simulink model "r2_b8a4x128f_4gbe"  (R2012b)
settings: Solver=VariableStepDiscrete  SolverMode=SingleTasking  StartTime=0.0  StopTime=1  RelTol=1e-3
undefined symbols (not defined in the file): fft_stages, n_ants, n_bits_xengs
libraries: xbsIndex_r4 x21845, casper_library_misc x157, xbsReplacements_r4 x24, casper_library_communications x8, casper_library_delays x8, xps_library x5
(part 15 of 182)

== system r2_b8a4x128f_4gbe/latch0 ==
  reset : Inport
  gbe_down : Inport  Port=2
  rx_dest_err : Inport  Port=3
  feng_rx_err : Inport  Port=4
  fft_err : Inport  Port=5
  feng_qdr_err : Inport  Port=6
  feng_chk_err : Inport  Port=7
  adc_over : Inport  Port=8
  noise_diode_en : Inport  Port=9
  vacc_err : Inport  Port=10
  rx_bad_pkt : Inport  Port=11
  rx_bad_frame : Inport  Port=12
  tx_over : Inport  Port=13
  xeng_bad_dat : Inport  Port=14
  pack_err : Inport  Port=15
  rx : Inport  Port=16
  tx : Inport  Port=17
  flush : Inport  Port=18
  Delay{,1..16,33} (18 alike) : xbsIndex_r4/Delay  rst=off  infoeditControl=Selection of Reset will increase slice count due to use of real FFs and instead of SRLs  en=off  latency=1  dbl_ovrd=off  reg_retiming=off  block_type=delay
  Delay{17..32,34} (17 alike) : xbsIndex_r4/Delay  rst=on  infoeditControl=Selection of Reset will increase slice count due to use of real FFs and instead of SRLs  en=on  latency=1  dbl_ovrd=off  reg_retiming=on  block_type=delay
  Subsystem6 : Subsystem
  gbe_down_reg : Outport
  rx_dest_err_reg : Outport  Port=2
  feng_rx_err_reg : Outport  Port=3
  fft_err_reg : Outport  Port=4
  feng_qdr_err_reg : Outport  Port=5
  feng_chk_err_reg : Outport  Port=6
  adc_over_reg : Outport  Port=7
  noise_diode_en_reg : Outport  Port=8
  vacc_err_reg : Outport  Port=9
  rx_bad_pkt_reg : Outport  Port=10
  rx_bad_frame_reg : Outport  Port=11
  tx_over_reg : Outport  Port=12
  xeng_bad_dat_reg : Outport  Port=13
  pack_err_reg : Outport  Port=14
  rx_reg : Outport  Port=15
  tx_reg : Outport  Port=16
  data_bad : Outport  Port=17
  error : Outport  Port=18
  flush_reg : Outport  Port=19
  wires:
  rx_bad_pkt/1 -> Delay10/1
  pack_err/1 -> Delay14/1
  xeng_bad_dat/1 -> Delay13/1
  tx_over/1 -> Delay12/1
  rx_bad_frame/1 -> Delay11/1
  vacc_err/1 -> Delay9/1
  noise_diode_en/1 -> Delay8/1
  adc_over/1 -> Delay7/1
  feng_chk_err/1 -> Delay6/1
  feng_qdr_err/1 -> Delay5/1
  Subsystem6/2(err) -> error/1
  Subsystem6/1(data_in_bad) -> data_bad/1
  fft_err/1 -> Delay4/1
  feng_rx_err/1 -> Delay3/1
  rx_dest_err/1 -> Delay2/1
  gbe_down/1 -> Delay1/1
  reset/1 -> Delay/1
  Delay28/1 -> tx_over_reg/1
  Delay27/1 -> rx_bad_frame_reg/1
  Delay26/1 -> rx_bad_pkt_reg/1
  Delay25/1 -> vacc_err_reg/1
  Delay24/1 -> noise_diode_en_reg/1
  Delay23/1 -> adc_over_reg/1
  Delay22/1 -> feng_chk_err_reg/1
  Delay21/1 -> feng_qdr_err_reg/1
  Delay20/1 -> fft_err_reg/1
  Delay19/1 -> feng_rx_err_reg/1
  Delay17/1 -> gbe_down_reg/1
  Delay18/1 -> rx_dest_err_reg/1
  rx/1 -> Delay15/1
  Delay31/1 -> rx_reg/1
  tx/1 -> Delay16/1
  Delay32/1 -> tx_reg/1
  Delay/1 -> Delay17/2, Delay18/2, Delay19/2, Delay20/2, Delay21/2, Delay22/2, Delay23/2, Delay24/2, Delay25/2, Delay26/2, Delay27/2, Delay28/2, Delay29/2, Delay30/2, Delay34/2, Delay32/2, Delay31/2
  Delay1/1 -> Subsystem6/1(gbe_down), Delay17/3, Delay17/1
  Delay2/1 -> Delay18/3, Delay18/1, Subsystem6/2(rx_dest_err)
  Delay3/1 -> Delay19/3, Delay19/1, Subsystem6/3(feng_rx_err)
  Delay4/1 -> Delay20/1, Delay20/3, Subsystem6/4(fft_err)
  Delay7/1 -> Delay23/1, Delay23/3, Subsystem6/7(adc_over)
  Delay6/1 -> Delay22/1, Delay22/3, Subsystem6/6(feng_chk_err)
  Delay5/1 -> Delay21/3, Delay21/1, Subsystem6/5(feng_qdr_err)
  Delay11/1 -> Delay27/3, Delay27/1, Subsystem6/10(rx_bad_frame)
  Delay15/1 -> Delay31/1, Delay31/3
  Delay9/1 -> Delay25/3, Delay25/1, Subsystem6/8(vacc_err)
  Delay8/1 -> Delay24/1, Delay24/3
  Delay10/1 -> Delay26/1, Delay26/3, Subsystem6/9(rx_bad_pkt)
  Delay12/1 -> Delay28/1, Delay28/3, Subsystem6/11(tx_over)
  Delay13/1 -> Delay29/1, Delay29/3, Subsystem6/12(xeng_bad_dat)
  Delay14/1 -> Delay30/3, Delay30/1, Subsystem6/13(pack_err)
  Delay16/1 -> Delay32/3, Delay32/1
  Delay29/1 -> xeng_bad_dat_reg/1
  Delay30/1 -> pack_err_reg/1
  flush/1 -> Delay33/1
  Delay33/1 -> Delay34/3, Delay34/1
  Delay34/1 -> flush_reg/1

== system r2_b8a4x128f_4gbe/latch1 ==
  reset : Inport
  gbe_down : Inport  Port=2
  rx_dest_err : Inport  Port=3
  feng_rx_err : Inport  Port=4
  fft_err : Inport  Port=5
  feng_qdr_err : Inport  Port=6
  feng_chk_err : Inport  Port=7
  adc_over : Inport  Port=8
  noise_diode_en : Inport  Port=9
  vacc_err : Inport  Port=10
  rx_bad_pkt : Inport  Port=11
  rx_bad_frame : Inport  Port=12
  tx_over : Inport  Port=13
  xeng_bad_dat : Inport  Port=14
  pack_err : Inport  Port=15
  rx : Inport  Port=16
  tx : Inport  Port=17
  flush : Inport  Port=18
  Delay{,1..16,33} (18 alike) : xbsIndex_r4/Delay  rst=off  infoeditControl=Selection of Reset will increase slice count due to use of real FFs and instead of SRLs  en=off  latency=1  dbl_ovrd=off  reg_retiming=off  block_type=delay
  Delay{17..32,34} (17 alike) : xbsIndex_r4/Delay  rst=on  infoeditControl=Selection of Reset will increase slice count due to use of real FFs and instead of SRLs  en=on  latency=1  dbl_ovrd=off  reg_retiming=on  block_type=delay
  Subsystem6 : Subsystem
  gbe_down_reg : Outport
  rx_dest_err_reg : Outport  Port=2
  feng_rx_err_reg : Outport  Port=3
  fft_err_reg : Outport  Port=4
  feng_qdr_err_reg : Outport  Port=5
  feng_chk_err_reg : Outport  Port=6
  adc_over_reg : Outport  Port=7
  noise_diode_en_reg : Outport  Port=8
  vacc_err_reg : Outport  Port=9
  rx_bad_pkt_reg : Outport  Port=10
  rx_bad_frame_reg : Outport  Port=11
  tx_over_reg : Outport  Port=12
  xeng_bad_dat_reg : Outport  Port=13
  pack_err_reg : Outport  Port=14
  rx_reg : Outport  Port=15
  tx_reg : Outport  Port=16
  data_bad : Outport  Port=17
  error : Outport  Port=18
  flush_reg : Outport  Port=19
  wires:
  Delay34/1 -> flush_reg/1
  Delay33/1 -> Delay34/1, Delay34/3
  flush/1 -> Delay33/1
  Delay30/1 -> pack_err_reg/1
  Delay29/1 -> xeng_bad_dat_reg/1
  Delay16/1 -> Delay32/1, Delay32/3
  Delay14/1 -> Subsystem6/13(pack_err), Delay30/1, Delay30/3
  Delay13/1 -> Subsystem6/12(xeng_bad_dat), Delay29/3, Delay29/1
  Delay12/1 -> Subsystem6/11(tx_over), Delay28/3, Delay28/1
  Delay10/1 -> Subsystem6/9(rx_bad_pkt), Delay26/3, Delay26/1
  Delay8/1 -> Delay24/3, Delay24/1
  Delay9/1 -> Subsystem6/8(vacc_err), Delay25/1, Delay25/3
  Delay15/1 -> Delay31/3, Delay31/1
  Delay11/1 -> Subsystem6/10(rx_bad_frame), Delay27/1, Delay27/3
  Delay5/1 -> Subsystem6/5(feng_qdr_err), Delay21/1, Delay21/3
  Delay6/1 -> Subsystem6/6(feng_chk_err), Delay22/3, Delay22/1
  Delay7/1 -> Subsystem6/7(adc_over), Delay23/3, Delay23/1
  Delay4/1 -> Subsystem6/4(fft_err), Delay20/3, Delay20/1
  Delay3/1 -> Subsystem6/3(feng_rx_err), Delay19/1, Delay19/3
  Delay2/1 -> Subsystem6/2(rx_dest_err), Delay18/1, Delay18/3
  Delay1/1 -> Delay17/1, Delay17/3, Subsystem6/1(gbe_down)
  Delay/1 -> Delay31/2, Delay32/2, Delay34/2, Delay30/2, Delay29/2, Delay28/2, Delay27/2, Delay26/2, Delay25/2, Delay24/2, Delay23/2, Delay22/2, Delay21/2, Delay20/2, Delay19/2, Delay18/2, Delay17/2
  Delay32/1 -> tx_reg/1
  tx/1 -> Delay16/1
  Delay31/1 -> rx_reg/1
  rx/1 -> Delay15/1
  Delay18/1 -> rx_dest_err_reg/1
  Delay17/1 -> gbe_down_reg/1
  Delay19/1 -> feng_rx_err_reg/1
  Delay20/1 -> fft_err_reg/1
  Delay21/1 -> feng_qdr_err_reg/1
  Delay22/1 -> feng_chk_err_reg/1
  Delay23/1 -> adc_over_reg/1
  Delay24/1 -> noise_diode_en_reg/1
  Delay25/1 -> vacc_err_reg/1
  Delay26/1 -> rx_bad_pkt_reg/1
  Delay27/1 -> rx_bad_frame_reg/1
  Delay28/1 -> tx_over_reg/1
  reset/1 -> Delay/1
  gbe_down/1 -> Delay1/1
  rx_dest_err/1 -> Delay2/1
  feng_rx_err/1 -> Delay3/1
  fft_err/1 -> Delay4/1
  Subsystem6/1(data_in_bad) -> data_bad/1
  Subsystem6/2(err) -> error/1
  feng_qdr_err/1 -> Delay5/1
  feng_chk_err/1 -> Delay6/1
  adc_over/1 -> Delay7/1
  noise_diode_en/1 -> Delay8/1
  vacc_err/1 -> Delay9/1
  rx_bad_frame/1 -> Delay11/1
  tx_over/1 -> Delay12/1
  xeng_bad_dat/1 -> Delay13/1
  pack_err/1 -> Delay14/1
  rx_bad_pkt/1 -> Delay10/1

== system r2_b8a4x128f_4gbe/latch2 ==
  reset : Inport
  gbe_down : Inport  Port=2
  rx_dest_err : Inport  Port=3
  feng_rx_err : Inport  Port=4
  fft_err : Inport  Port=5
  feng_qdr_err : Inport  Port=6
  feng_chk_err : Inport  Port=7
  adc_over : Inport  Port=8
  noise_diode_en : Inport  Port=9
  vacc_err : Inport  Port=10
  rx_bad_pkt : Inport  Port=11
  rx_bad_frame : Inport  Port=12
  tx_over : Inport  Port=13
  xeng_bad_dat : Inport  Port=14
  pack_err : Inport  Port=15
  rx : Inport  Port=16
  tx : Inport  Port=17
  flush : Inport  Port=18
  Delay{,1..16,33} (18 alike) : xbsIndex_r4/Delay  rst=off  infoeditControl=Selection of Reset will increase slice count due to use of real FFs and instead of SRLs  en=off  latency=1  dbl_ovrd=off  reg_retiming=off  block_type=delay
  Delay{17..32,34} (17 alike) : xbsIndex_r4/Delay  rst=on  infoeditControl=Selection of Reset will increase slice count due to use of real FFs and instead of SRLs  en=on  latency=1  dbl_ovrd=off  reg_retiming=on  block_type=delay
  Subsystem6 : Subsystem
  gbe_down_reg : Outport
  rx_dest_err_reg : Outport  Port=2
  feng_rx_err_reg : Outport  Port=3
  fft_err_reg : Outport  Port=4
  feng_qdr_err_reg : Outport  Port=5
  feng_chk_err_reg : Outport  Port=6
  adc_over_reg : Outport  Port=7
  noise_diode_en_reg : Outport  Port=8
  vacc_err_reg : Outport  Port=9
  rx_bad_pkt_reg : Outport  Port=10
  rx_bad_frame_reg : Outport  Port=11
  tx_over_reg : Outport  Port=12
  xeng_bad_dat_reg : Outport  Port=13
  pack_err_reg : Outport  Port=14
  rx_reg : Outport  Port=15
  tx_reg : Outport  Port=16
  data_bad : Outport  Port=17
  error : Outport  Port=18
  flush_reg : Outport  Port=19
  wires:
  rx_bad_pkt/1 -> Delay10/1
  pack_err/1 -> Delay14/1
  xeng_bad_dat/1 -> Delay13/1
  tx_over/1 -> Delay12/1
  rx_bad_frame/1 -> Delay11/1
  vacc_err/1 -> Delay9/1
  noise_diode_en/1 -> Delay8/1
  adc_over/1 -> Delay7/1
  feng_chk_err/1 -> Delay6/1
  feng_qdr_err/1 -> Delay5/1
  Subsystem6/2(err) -> error/1
  Subsystem6/1(data_in_bad) -> data_bad/1
  fft_err/1 -> Delay4/1
  feng_rx_err/1 -> Delay3/1
  rx_dest_err/1 -> Delay2/1
  gbe_down/1 -> Delay1/1
  reset/1 -> Delay/1
  Delay28/1 -> tx_over_reg/1
  Delay27/1 -> rx_bad_frame_reg/1
  Delay26/1 -> rx_bad_pkt_reg/1
  Delay25/1 -> vacc_err_reg/1
  Delay24/1 -> noise_diode_en_reg/1
  Delay23/1 -> adc_over_reg/1
  Delay22/1 -> feng_chk_err_reg/1
  Delay21/1 -> feng_qdr_err_reg/1
  Delay20/1 -> fft_err_reg/1
  Delay19/1 -> feng_rx_err_reg/1
  Delay17/1 -> gbe_down_reg/1
  Delay18/1 -> rx_dest_err_reg/1
  rx/1 -> Delay15/1
  Delay31/1 -> rx_reg/1
  tx/1 -> Delay16/1
  Delay32/1 -> tx_reg/1
  Delay/1 -> Delay17/2, Delay18/2, Delay19/2, Delay20/2, Delay21/2, Delay22/2, Delay23/2, Delay24/2, Delay25/2, Delay26/2, Delay27/2, Delay28/2, Delay29/2, Delay30/2, Delay34/2, Delay32/2, Delay31/2
  Delay1/1 -> Subsystem6/1(gbe_down), Delay17/3, Delay17/1
  Delay2/1 -> Delay18/3, Delay18/1, Subsystem6/2(rx_dest_err)
  Delay3/1 -> Delay19/3, Delay19/1, Subsystem6/3(feng_rx_err)
  Delay4/1 -> Delay20/1, Delay20/3, Subsystem6/4(fft_err)
  Delay7/1 -> Delay23/1, Delay23/3, Subsystem6/7(adc_over)
  Delay6/1 -> Delay22/1, Delay22/3, Subsystem6/6(feng_chk_err)
  Delay5/1 -> Delay21/3, Delay21/1, Subsystem6/5(feng_qdr_err)
  Delay11/1 -> Delay27/3, Delay27/1, Subsystem6/10(rx_bad_frame)
  Delay15/1 -> Delay31/1, Delay31/3
  Delay9/1 -> Delay25/3, Delay25/1, Subsystem6/8(vacc_err)
  Delay8/1 -> Delay24/1, Delay24/3
  Delay10/1 -> Delay26/1, Delay26/3, Subsystem6/9(rx_bad_pkt)
  Delay12/1 -> Delay28/1, Delay28/3, Subsystem6/11(tx_over)
  Delay13/1 -> Delay29/1, Delay29/3, Subsystem6/12(xeng_bad_dat)
  Delay14/1 -> Delay30/3, Delay30/1, Subsystem6/13(pack_err)
  Delay16/1 -> Delay32/3, Delay32/1
  Delay29/1 -> xeng_bad_dat_reg/1
  Delay30/1 -> pack_err_reg/1
  flush/1 -> Delay33/1
  Delay33/1 -> Delay34/3, Delay34/1
  Delay34/1 -> flush_reg/1

== system r2_b8a4x128f_4gbe/latch3 ==
  reset : Inport
  gbe_down : Inport  Port=2
  rx_dest_err : Inport  Port=3
  feng_rx_err : Inport  Port=4
  fft_err : Inport  Port=5
  feng_qdr_err : Inport  Port=6
  feng_chk_err : Inport  Port=7
  adc_over : Inport  Port=8
  noise_diode_en : Inport  Port=9
  vacc_err : Inport  Port=10
  rx_bad_pkt : Inport  Port=11
  rx_bad_frame : Inport  Port=12
  tx_over : Inport  Port=13
  xeng_bad_dat : Inport  Port=14
  pack_err : Inport  Port=15
  rx : Inport  Port=16
  tx : Inport  Port=17
  flush : Inport  Port=18
  Delay{,1..16,33} (18 alike) : xbsIndex_r4/Delay  rst=off  infoeditControl=Selection of Reset will increase slice count due to use of real FFs and instead of SRLs  en=off  latency=1  dbl_ovrd=off  reg_retiming=off  block_type=delay
  Delay{17..32,34} (17 alike) : xbsIndex_r4/Delay  rst=on  infoeditControl=Selection of Reset will increase slice count due to use of real FFs and instead of SRLs  en=on  latency=1  dbl_ovrd=off  reg_retiming=on  block_type=delay
  Subsystem6 : Subsystem
  gbe_down_reg : Outport
  rx_dest_err_reg : Outport  Port=2
  feng_rx_err_reg : Outport  Port=3
  fft_err_reg : Outport  Port=4
  feng_qdr_err_reg : Outport  Port=5
  feng_chk_err_reg : Outport  Port=6
  adc_over_reg : Outport  Port=7
  noise_diode_en_reg : Outport  Port=8
  vacc_err_reg : Outport  Port=9
  rx_bad_pkt_reg : Outport  Port=10
  rx_bad_frame_reg : Outport  Port=11
  tx_over_reg : Outport  Port=12
  xeng_bad_dat_reg : Outport  Port=13
  pack_err_reg : Outport  Port=14
  rx_reg : Outport  Port=15
  tx_reg : Outport  Port=16
  data_bad : Outport  Port=17
  error : Outport  Port=18
  flush_reg : Outport  Port=19
  wires:
  Delay34/1 -> flush_reg/1
  Delay33/1 -> Delay34/1, Delay34/3
  flush/1 -> Delay33/1
  Delay30/1 -> pack_err_reg/1
  Delay29/1 -> xeng_bad_dat_reg/1
  Delay16/1 -> Delay32/1, Delay32/3
  Delay14/1 -> Subsystem6/13(pack_err), Delay30/1, Delay30/3
  Delay13/1 -> Subsystem6/12(xeng_bad_dat), Delay29/3, Delay29/1
  Delay12/1 -> Subsystem6/11(tx_over), Delay28/3, Delay28/1
  Delay10/1 -> Subsystem6/9(rx_bad_pkt), Delay26/3, Delay26/1
  Delay8/1 -> Delay24/3, Delay24/1
  Delay9/1 -> Subsystem6/8(vacc_err), Delay25/1, Delay25/3
  Delay15/1 -> Delay31/3, Delay31/1
  Delay11/1 -> Subsystem6/10(rx_bad_frame), Delay27/1, Delay27/3
  Delay5/1 -> Subsystem6/5(feng_qdr_err), Delay21/1, Delay21/3
  Delay6/1 -> Subsystem6/6(feng_chk_err), Delay22/3, Delay22/1
  Delay7/1 -> Subsystem6/7(adc_over), Delay23/3, Delay23/1
  Delay4/1 -> Subsystem6/4(fft_err), Delay20/3, Delay20/1
  Delay3/1 -> Subsystem6/3(feng_rx_err), Delay19/1, Delay19/3
  Delay2/1 -> Subsystem6/2(rx_dest_err), Delay18/1, Delay18/3
  Delay1/1 -> Delay17/1, Delay17/3, Subsystem6/1(gbe_down)
  Delay/1 -> Delay31/2, Delay32/2, Delay34/2, Delay30/2, Delay29/2, Delay28/2, Delay27/2, Delay26/2, Delay25/2, Delay24/2, Delay23/2, Delay22/2, Delay21/2, Delay20/2, Delay19/2, Delay18/2, Delay17/2
  Delay32/1 -> tx_reg/1
  tx/1 -> Delay16/1
  Delay31/1 -> rx_reg/1
  rx/1 -> Delay15/1
  Delay18/1 -> rx_dest_err_reg/1
  Delay17/1 -> gbe_down_reg/1
  Delay19/1 -> feng_rx_err_reg/1
  Delay20/1 -> fft_err_reg/1
  Delay21/1 -> feng_qdr_err_reg/1
  Delay22/1 -> feng_chk_err_reg/1
  Delay23/1 -> adc_over_reg/1
  Delay24/1 -> noise_diode_en_reg/1
  Delay25/1 -> vacc_err_reg/1
  Delay26/1 -> rx_bad_pkt_reg/1
  Delay27/1 -> rx_bad_frame_reg/1
  Delay28/1 -> tx_over_reg/1
  reset/1 -> Delay/1
  gbe_down/1 -> Delay1/1
  rx_dest_err/1 -> Delay2/1
  feng_rx_err/1 -> Delay3/1
  fft_err/1 -> Delay4/1
  Subsystem6/1(data_in_bad) -> data_bad/1
  Subsystem6/2(err) -> error/1
  feng_qdr_err/1 -> Delay5/1
  feng_chk_err/1 -> Delay6/1
  adc_over/1 -> Delay7/1
  noise_diode_en/1 -> Delay8/1
  vacc_err/1 -> Delay9/1
  rx_bad_frame/1 -> Delay11/1
  tx_over/1 -> Delay12/1
  xeng_bad_dat/1 -> Delay13/1
  pack_err/1 -> Delay14/1
  rx_bad_pkt/1 -> Delay10/1

== system r2_b8a4x128f_4gbe/miss_cnt0 ==
  Convert : xbsIndex_r4/Convert  gui_display_data_type=Fixed-point  arith_type=Unsigned  n_bits=32  bin_pt=0  float_type=Single  exp_bits=8  fraction_bits=24  quantization=Truncate  overflow=Wrap  en=off  latency=0  dbl_ovrd=off  pipeline=off  block_type=convert
  Counter1 : xbsIndex_r4/Counter  cnt_type=Free Running  cnt_to=1023  operation=Up  start_count=0  cnt_by_val=1  arith_type=Unsigned  n_bits=16  bin_pt=0  load_pin=off  rst=on  en=on  explicit_period=on  period=1  dbl_ovrd=off  use_behavioral_HDL=on  implementation=Fabric  use_rpm=on  block_type=counter
      settings: xl_area=[0, 0, 0, 0, 0, 0, 0]
  Delay1 : Subsystem  AncestorBlock=casper_library_delays/pipeline  mask(pipeline){latency=2}
      mask help:
      | An explicitly laid-out delay line to avoid mapping to SRL16s
      | for use in pipelining to help achieve timing closure.
      mask init:
      | pipeline_init(gcb,'latency',latency);
      settings: AttributesFormatString=Latency = %<latency>
      mask Display:
      | port_label('input', 1, 'd');
      | port_label('output', 1, 'q');
      | disp(['Z^-', num2str(latency)]);
  Delay10 : Subsystem  AncestorBlock=casper_library_delays/pipeline  mask(pipeline){latency=2}
      mask help:
      | An explicitly laid-out delay line to avoid mapping to SRL16s
      | for use in pipelining to help achieve timing closure.
      mask init:
      | pipeline_init(gcb,'latency',latency);
      settings: AttributesFormatString=Latency = %<latency>
      mask Display:
      | port_label('input', 1, 'd');
      | port_label('output', 1, 'q');
      | disp(['Z^-', num2str(latency)]);
  Delay11 : Subsystem  AncestorBlock=casper_library_delays/pipeline  mask(pipeline){latency=2}
      mask help:
      | An explicitly laid-out delay line to avoid mapping to SRL16s
      | for use in pipelining to help achieve timing closure.
      mask init:
      | pipeline_init(gcb,'latency',latency);
      settings: AttributesFormatString=Latency = %<latency>
      mask Display:
      | port_label('input', 1, 'd');
      | port_label('output', 1, 'q');
      | disp(['Z^-', num2str(latency)]);
  Delay12 : Subsystem  AncestorBlock=casper_library_delays/pipeline  mask(pipeline){latency=2}
      mask help:
      | An explicitly laid-out delay line to avoid mapping to SRL16s
      | for use in pipelining to help achieve timing closure.
      mask init:
      | pipeline_init(gcb,'latency',latency);
      settings: AttributesFormatString=Latency = %<latency>
      mask Display:
      | port_label('input', 1, 'd');
      | port_label('output', 1, 'q');
      | disp(['Z^-', num2str(latency)]);
  Delay13 : Subsystem  AncestorBlock=casper_library_delays/pipeline  mask(pipeline){latency=2}
      mask help:
      | An explicitly laid-out delay line to avoid mapping to SRL16s
      | for use in pipelining to help achieve timing closure.
      mask init:
      | pipeline_init(gcb,'latency',latency);
      settings: AttributesFormatString=Latency = %<latency>
      mask Display:
      | port_label('input', 1, 'd');
      | port_label('output', 1, 'q');
      | disp(['Z^-', num2str(latency)]);
  Delay14 : Subsystem  AncestorBlock=casper_library_delays/pipeline  mask(pipeline){latency=2}
      mask help:
      | An explicitly laid-out delay line to avoid mapping to SRL16s
      | for use in pipelining to help achieve timing closure.
      mask init:
      | pipeline_init(gcb,'latency',latency);
      settings: AttributesFormatString=Latency = %<latency>
      mask Display:
      | port_label('input', 1, 'd');
      | port_label('output', 1, 'q');
      | disp(['Z^-', num2str(latency)]);
  Delay15 : Subsystem  AncestorBlock=casper_library_delays/pipeline  mask(pipeline){latency=2}
      mask help:
      | An explicitly laid-out delay line to avoid mapping to SRL16s
      | for use in pipelining to help achieve timing closure.
      mask init:
      | pipeline_init(gcb,'latency',latency);
      settings: AttributesFormatString=Latency = %<latency>
      mask Display:
      | port_label('input', 1, 'd');
      | port_label('output', 1, 'q');
      | disp(['Z^-', num2str(latency)]);
  Delay2 : Subsystem  AncestorBlock=casper_library_delays/pipeline  mask(pipeline){latency=2}
      mask help:
      | An explicitly laid-out delay line to avoid mapping to SRL16s
      | for use in pipelining to help achieve timing closure.
      mask init:
      | pipeline_init(gcb,'latency',latency);
      settings: AttributesFormatString=Latency = %<latency>
      mask Display:
      | port_label('input', 1, 'd');
      | port_label('output', 1, 'q');
      | disp(['Z^-', num2str(latency)]);
  Delay3 : Subsystem  AncestorBlock=casper_library_delays/pipeline  mask(pipeline){latency=2}
      mask help:
      | An explicitly laid-out delay line to avoid mapping to SRL16s
      | for use in pipelining to help achieve timing closure.
      mask init:
      | pipeline_init(gcb,'latency',latency);
      settings: AttributesFormatString=Latency = %<latency>
      mask Display:
      | port_label('input', 1, 'd');
      | port_label('output', 1, 'q');
      | disp(['Z^-', num2str(latency)]);
  Delay4 : Subsystem  AncestorBlock=casper_library_delays/pipeline  mask(pipeline){latency=1}
      mask help:
      | An explicitly laid-out delay line to avoid mapping to SRL16s
      | for use in pipelining to help achieve timing closure.
      mask init:
      | pipeline_init(gcb,'latency',latency);
      settings: AttributesFormatString=Latency = %<latency>
      mask Display:
      | port_label('input', 1, 'd');
      | port_label('output', 1, 'q');
      | disp(['Z^-', num2str(latency)]);
  Delay5 : Subsystem  AncestorBlock=casper_library_delays/pipeline  mask(pipeline){latency=2}
      mask help:
      | An explicitly laid-out delay line to avoid mapping to SRL16s
      | for use in pipelining to help achieve timing closure.
      mask init:
      | pipeline_init(gcb,'latency',latency);
      settings: AttributesFormatString=Latency = %<latency>
      mask Display:
      | port_label('input', 1, 'd');
      | port_label('output', 1, 'q');
      | disp(['Z^-', num2str(latency)]);
  Delay6 : Subsystem  AncestorBlock=casper_library_delays/pipeline  mask(pipeline){latency=3}
      mask help:
      | An explicitly laid-out delay line to avoid mapping to SRL16s
      | for use in pipelining to help achieve timing closure.
      mask init:
      | pipeline_init(gcb,'latency',latency);
      settings: AttributesFormatString=Latency = %<latency>
      mask Display:
      | port_label('input', 1, 'd');
      | port_label('output', 1, 'q');
      | disp(['Z^-', num2str(latency)]);
  Delay7 : Subsystem  AncestorBlock=casper_library_delays/pipeline  mask(pipeline){latency=2}
      mask help:
      | An explicitly laid-out delay line to avoid mapping to SRL16s
      | for use in pipelining to help achieve timing closure.
      mask init:
      | pipeline_init(gcb,'latency',latency);
      settings: AttributesFormatString=Latency = %<latency>
      mask Display:
      | port_label('input', 1, 'd');
      | port_label('output', 1, 'q');
      | disp(['Z^-', num2str(latency)]);
  Delay8 : Subsystem  AncestorBlock=casper_library_delays/pipeline  mask(pipeline){latency=2}
      mask help:
      | An explicitly laid-out delay line to avoid mapping to SRL16s
      | for use in pipelining to help achieve timing closure.
      mask init:
      | pipeline_init(gcb,'latency',latency);
      settings: AttributesFormatString=Latency = %<latency>
      mask Display:
      | port_label('input', 1, 'd');
      | port_label('output', 1, 'q');
      | disp(['Z^-', num2str(latency)]);
  Delay9 : Subsystem  AncestorBlock=casper_library_delays/pipeline  mask(pipeline){latency=2}
      mask help:
      | An explicitly laid-out delay line to avoid mapping to SRL16s
      | for use in pipelining to help achieve timing closure.
      mask init:
      | pipeline_init(gcb,'latency',latency);
      settings: AttributesFormatString=Latency = %<latency>
      mask Display:
      | port_label('input', 1, 'd');
      | port_label('output', 1, 'q');
      | disp(['Z^-', num2str(latency)]);
  Delay96 : Subsystem  AncestorBlock=casper_library_delays/pipeline  mask(pipeline){latency=2}
      mask help:
      | An explicitly laid-out delay line to avoid mapping to SRL16s
      | for use in pipelining to help achieve timing closure.
      mask init:
      | pipeline_init(gcb,'latency',latency);
      settings: AttributesFormatString=Latency = %<latency>
      mask Display:
      | port_label('input', 1, 'd');
      | port_label('output', 1, 'q');
      | disp(['Z^-', num2str(latency)]);
  Delay97 : Subsystem  AncestorBlock=casper_library_delays/pipeline  mask(pipeline){latency=2}
      mask help:
      | An explicitly laid-out delay line to avoid mapping to SRL16s
      | for use in pipelining to help achieve timing closure.
      mask init:
      | pipeline_init(gcb,'latency',latency);
      settings: AttributesFormatString=Latency = %<latency>
      mask Display:
      | port_label('input', 1, 'd');
      | port_label('output', 1, 'q');
      | disp(['Z^-', num2str(latency)]);
  Delay98 : Subsystem  AncestorBlock=casper_library_delays/pipeline  mask(pipeline){latency=2}
      mask help:
      | An explicitly laid-out delay line to avoid mapping to SRL16s
      | for use in pipelining to help achieve timing closure.
      mask init:
      | pipeline_init(gcb,'latency',latency);
      settings: AttributesFormatString=Latency = %<latency>
      mask Display:
      | port_label('input', 1, 'd');
      | port_label('output', 1, 'q');
      | disp(['Z^-', num2str(latency)]);
  Logical{1..4} (4 alike) : xbsIndex_r4/Logical  logical_function=AND  inputs=2  en=off  latency=1  precision=Full  arith_type=Unsigned  n_bits=8  bin_pt=2  align_bp=on  dbl_ovrd=off  block_type=logical
      settings: xl_area=[0, 0, 0, 0, 0, 0, 0]
  Register : xbsIndex_r4/Register  init=0  rst=on  en=on  dbl_ovrd=off  block_type=register
  Slice : xbsIndex_r4/Slice  nbits=16  boolean_output=off  mode=Two Bit Locations  bit1=0  base1=MSB of Input  bit0=xeng_int_bits  base0=LSB of Input  dbl_ovrd=off  block_type=slice
      settings: infoedit="Extracts a given range of bits from each input sample and presents it at the output.  The output type is ordinarily unsigned with binary point at zero, but can be Boolean when the slice is one bit wide.<P><P>Hardware notes: In hardware this block costs nothing."  block_version=10.1.3
  ant_cnt : xbsIndex_r4/Counter  cnt_type=Free Running  cnt_to=1023  operation=Up  start_count=0  cnt_by_val=1  arith_type=Unsigned  n_bits=xeng_int_bits + n_ants_bits  bin_pt=0  load_pin=off  rst=on  en=on  explicit_period=on  period=1  dbl_ovrd=off  use_behavioral_HDL=on  implementation=Fabric  use_rpm=on  block_type=counter
      settings: xl_area=[0, 0, 0, 0, 0, 0, 0]
  sync_ctr1 : xbsIndex_r4/Counter  cnt_type=Free Running  cnt_to=1023  operation=Up  start_count=0  cnt_by_val=1  arith_type=Unsigned  n_bits=32  bin_pt=0  load_pin=off  rst=on  en=on  explicit_period=on  period=1  dbl_ovrd=off  use_behavioral_HDL=off  implementation=Fabric  use_rpm=on  block_type=counter
      settings: xl_area=[0, 0, 0, 0, 0, 0, 0]
  sync_ctr5 : xbsIndex_r4/Counter  cnt_type=Free Running  cnt_to=1023  operation=Up  start_count=0  cnt_by_val=1  arith_type=Unsigned  n_bits=16  bin_pt=0  load_pin=off  rst=on  en=on  explicit_period=on  period=1  dbl_ovrd=off  use_behavioral_HDL=on  implementation=Fabric  use_rpm=on  block_type=counter
      settings: xl_area=[0, 0, 0, 0, 0, 0, 0]
  sync_ctr6 : xbsIndex_r4/Counter  cnt_type=Free Running  cnt_to=1023  operation=Up  start_count=0  cnt_by_val=1  arith_type=Unsigned  n_bits=16  bin_pt=0  load_pin=off  rst=on  en=on  explicit_period=on  period=1  dbl_ovrd=off  use_behavioral_HDL=on  implementation=Fabric  use_rpm=on  block_type=counter
      settings: xl_area=[0, 0, 0, 0, 0, 0, 0]
  sync_ctr8 : xbsIndex_r4/Counter  cnt_type=Free Running  cnt_to=1023  operation=Up  start_count=0  cnt_by_val=1  arith_type=Unsigned  n_bits=32  bin_pt=0  load_pin=off  rst=on  en=on  explicit_period=on  period=1  dbl_ovrd=off  use_behavioral_HDL=off  implementation=Fabric  use_rpm=on  block_type=counter
      settings: xl_area=[0, 0, 0, 0, 0, 0, 0]
  spectr_cnt : Outport
  last_missed_ant : Outport  Port=2
  recv_ctr : Outport  Port=3
  recv_errctr : Outport  Port=4
  timeout_errctr : Outport  Port=5
  pktdisc_errctr : Outport  Port=6
  wires:
  Delay1/1(q) -> Register/2, Counter1/1
  Delay3/1(q) -> ant_cnt/2
  Delay2/1(q) -> Counter1/2, ant_cnt/1
  Counter1/1 -> Delay11/1(d)
  Register/1 -> Delay15/1(d)
  ant_cnt/1 -> Slice/1
  Slice/1 -> Register/1
  [reord_timeouterr0] -> Delay97/1(d)
  Logical3/1 -> sync_ctr6/2
  Delay96/1(q) -> sync_ctr1/1, sync_ctr5/1, sync_ctr6/1
  Delay97/1(q) -> Logical3/2
  [cnt_rst] -> Delay96/1(d)
  [reord_valid0] -> Delay98/1(d)
  Delay98/1(q) -> Logical2/1, Logical1/1, Logical3/1
  Logical1/1 -> sync_ctr5/2
  Delay8/1(q) -> Logical1/2
  [reord_pktdisc0] -> Delay8/1(d)
  sync_ctr8/1 -> Delay10/1(d)
  Logical4/1 -> sync_ctr8/2
  Delay12/1(q) -> sync_ctr8/1
  Delay13/1(q) -> Logical4/2
  [cnt_rst] -> Delay12/1(d)
  [reord_valid0] -> Delay14/1(d)
  Delay14/1(q) -> Logical4/1
  [reord_recv0] -> Delay13/1(d)
  sync_ctr6/1 -> Delay5/1(d)
  sync_ctr5/1 -> Delay6/1(d)
  sync_ctr1/1 -> Delay4/1(d)
  Delay4/1(q) -> recv_errctr/1
  Delay5/1(q) -> timeout_errctr/1
  Delay6/1(q) -> pktdisc_errctr/1
  Logical2/1 -> sync_ctr1/2
  Delay7/1(q) -> Logical2/2
  [reord_recverr0] -> Delay7/1(d)
  [cnt_rst] -> Delay1/1(d)
  [reord_sync0] -> Delay2/1(d)
  [reord_valid0] -> Delay3/1(d)
  [reord_recverr0] -> Delay9/1(d)
  Delay10/1(q) -> recv_ctr/1
  Delay11/1(q) -> spectr_cnt/1
  Delay15/1(q) -> Convert/1
  Convert/1 -> last_missed_ant/1
  Delay9/1(q) -> Register/3

== system r2_b8a4x128f_4gbe/miss_cnt1 ==
  Convert : xbsIndex_r4/Convert  gui_display_data_type=Fixed-point  arith_type=Unsigned  n_bits=32  bin_pt=0  float_type=Single  exp_bits=8  fraction_bits=24  quantization=Truncate  overflow=Wrap  en=off  latency=0  dbl_ovrd=off  pipeline=off  block_type=convert
  Counter1 : xbsIndex_r4/Counter  cnt_type=Free Running  cnt_to=1023  operation=Up  start_count=0  cnt_by_val=1  arith_type=Unsigned  n_bits=16  bin_pt=0  load_pin=off  rst=on  en=on  explicit_period=on  period=1  dbl_ovrd=off  use_behavioral_HDL=on  implementation=Fabric  use_rpm=on  block_type=counter
      settings: xl_area=[0, 0, 0, 0, 0, 0, 0]
  Delay1 : Subsystem  AncestorBlock=casper_library_delays/pipeline  mask(pipeline){latency=2}
      mask help:
      | An explicitly laid-out delay line to avoid mapping to SRL16s
      | for use in pipelining to help achieve timing closure.
      mask init:
      | pipeline_init(gcb,'latency',latency);
      settings: AttributesFormatString=Latency = %<latency>
      mask Display:
      | port_label('input', 1, 'd');
      | port_label('output', 1, 'q');
      | disp(['Z^-', num2str(latency)]);
  Delay10 : Subsystem  AncestorBlock=casper_library_delays/pipeline  mask(pipeline){latency=2}
      mask help:
      | An explicitly laid-out delay line to avoid mapping to SRL16s
      | for use in pipelining to help achieve timing closure.
      mask init:
      | pipeline_init(gcb,'latency',latency);
      settings: AttributesFormatString=Latency = %<latency>
      mask Display:
      | port_label('input', 1, 'd');
      | port_label('output', 1, 'q');
      | disp(['Z^-', num2str(latency)]);
  Delay11 : Subsystem  AncestorBlock=casper_library_delays/pipeline  mask(pipeline){latency=2}
      mask help:
      | An explicitly laid-out delay line to avoid mapping to SRL16s
      | for use in pipelining to help achieve timing closure.
      mask init:
      | pipeline_init(gcb,'latency',latency);
      settings: AttributesFormatString=Latency = %<latency>
      mask Display:
      | port_label('input', 1, 'd');
      | port_label('output', 1, 'q');
      | disp(['Z^-', num2str(latency)]);
  Delay12 : Subsystem  AncestorBlock=casper_library_delays/pipeline  mask(pipeline){latency=2}
      mask help:
      | An explicitly laid-out delay line to avoid mapping to SRL16s
      | for use in pipelining to help achieve timing closure.
      mask init:
      | pipeline_init(gcb,'latency',latency);
      settings: AttributesFormatString=Latency = %<latency>
      mask Display:
      | port_label('input', 1, 'd');
      | port_label('output', 1, 'q');
      | disp(['Z^-', num2str(latency)]);
  Delay13 : Subsystem  AncestorBlock=casper_library_delays/pipeline  mask(pipeline){latency=2}
      mask help:
      | An explicitly laid-out delay line to avoid mapping to SRL16s
      | for use in pipelining to help achieve timing closure.
      mask init:
      | pipeline_init(gcb,'latency',latency);
      settings: AttributesFormatString=Latency = %<latency>
      mask Display:
      | port_label('input', 1, 'd');
      | port_label('output', 1, 'q');
      | disp(['Z^-', num2str(latency)]);
  Delay14 : Subsystem  AncestorBlock=casper_library_delays/pipeline  mask(pipeline){latency=2}
      mask help:
      | An explicitly laid-out delay line to avoid mapping to SRL16s
      | for use in pipelining to help achieve timing closure.
      mask init:
      | pipeline_init(gcb,'latency',latency);
      settings: AttributesFormatString=Latency = %<latency>
      mask Display:
      | port_label('input', 1, 'd');
      | port_label('output', 1, 'q');
      | disp(['Z^-', num2str(latency)]);
  Delay15 : Subsystem  AncestorBlock=casper_library_delays/pipeline  mask(pipeline){latency=2}
      mask help:
      | An explicitly laid-out delay line to avoid mapping to SRL16s
      | for use in pipelining to help achieve timing closure.
      mask init:
      | pipeline_init(gcb,'latency',latency);
      settings: AttributesFormatString=Latency = %<latency>
      mask Display:
      | port_label('input', 1, 'd');
      | port_label('output', 1, 'q');
      | disp(['Z^-', num2str(latency)]);
  Delay2 : Subsystem  AncestorBlock=casper_library_delays/pipeline  mask(pipeline){latency=2}
      mask help:
      | An explicitly laid-out delay line to avoid mapping to SRL16s
      | for use in pipelining to help achieve timing closure.
      mask init:
      | pipeline_init(gcb,'latency',latency);
      settings: AttributesFormatString=Latency = %<latency>
      mask Display:
      | port_label('input', 1, 'd');
      | port_label('output', 1, 'q');
      | disp(['Z^-', num2str(latency)]);
  Delay3 : Subsystem  AncestorBlock=casper_library_delays/pipeline  mask(pipeline){latency=2}
      mask help:
      | An explicitly laid-out delay line to avoid mapping to SRL16s
      | for use in pipelining to help achieve timing closure.
      mask init:
      | pipeline_init(gcb,'latency',latency);
      settings: AttributesFormatString=Latency = %<latency>
      mask Display:
      | port_label('input', 1, 'd');
      | port_label('output', 1, 'q');
      | disp(['Z^-', num2str(latency)]);
  Delay4 : Subsystem  AncestorBlock=casper_library_delays/pipeline  mask(pipeline){latency=1}
      mask help:
      | An explicitly laid-out delay line to avoid mapping to SRL16s
      | for use in pipelining to help achieve timing closure.
      mask init:
      | pipeline_init(gcb,'latency',latency);
      settings: AttributesFormatString=Latency = %<latency>
      mask Display:
      | port_label('input', 1, 'd');
      | port_label('output', 1, 'q');
      | disp(['Z^-', num2str(latency)]);
  Delay5 : Subsystem  AncestorBlock=casper_library_delays/pipeline  mask(pipeline){latency=2}
      mask help:
      | An explicitly laid-out delay line to avoid mapping to SRL16s
      | for use in pipelining to help achieve timing closure.
      mask init:
      | pipeline_init(gcb,'latency',latency);
      settings: AttributesFormatString=Latency = %<latency>
      mask Display:
      | port_label('input', 1, 'd');
      | port_label('output', 1, 'q');
      | disp(['Z^-', num2str(latency)]);
  Delay6 : Subsystem  AncestorBlock=casper_library_delays/pipeline  mask(pipeline){latency=3}
      mask help:
      | An explicitly laid-out delay line to avoid mapping to SRL16s
      | for use in pipelining to help achieve timing closure.
      mask init:
      | pipeline_init(gcb,'latency',latency);
      settings: AttributesFormatString=Latency = %<latency>
      mask Display:
      | port_label('input', 1, 'd');
      | port_label('output', 1, 'q');
      | disp(['Z^-', num2str(latency)]);
  Delay7 : Subsystem  AncestorBlock=casper_library_delays/pipeline  mask(pipeline){latency=2}
      mask help:
      | An explicitly laid-out delay line to avoid mapping to SRL16s
      | for use in pipelining to help achieve timing closure.
      mask init:
      | pipeline_init(gcb,'latency',latency);
      settings: AttributesFormatString=Latency = %<latency>
      mask Display:
      | port_label('input', 1, 'd');
      | port_label('output', 1, 'q');
      | disp(['Z^-', num2str(latency)]);
  Delay8 : Subsystem  AncestorBlock=casper_library_delays/pipeline  mask(pipeline){latency=2}
      mask help:
      | An explicitly laid-out delay line to avoid mapping to SRL16s
      | for use in pipelining to help achieve timing closure.
      mask init:
      | pipeline_init(gcb,'latency',latency);
      settings: AttributesFormatString=Latency = %<latency>
      mask Display:
      | port_label('input', 1, 'd');
      | port_label('output', 1, 'q');
      | disp(['Z^-', num2str(latency)]);
  Delay9 : Subsystem  AncestorBlock=casper_library_delays/pipeline  mask(pipeline){latency=2}
      mask help:
      | An explicitly laid-out delay line to avoid mapping to SRL16s
      | for use in pipelining to help achieve timing closure.
      mask init:
      | pipeline_init(gcb,'latency',latency);
      settings: AttributesFormatString=Latency = %<latency>
      mask Display:
      | port_label('input', 1, 'd');
      | port_label('output', 1, 'q');
      | disp(['Z^-', num2str(latency)]);
  Delay96 : Subsystem  AncestorBlock=casper_library_delays/pipeline  mask(pipeline){latency=2}
      mask help:
      | An explicitly laid-out delay line to avoid mapping to SRL16s
      | for use in pipelining to help achieve timing closure.
      mask init:
      | pipeline_init(gcb,'latency',latency);
      settings: AttributesFormatString=Latency = %<latency>
      mask Display:
      | port_label('input', 1, 'd');
      | port_label('output', 1, 'q');
      | disp(['Z^-', num2str(latency)]);
  Delay97 : Subsystem  AncestorBlock=casper_library_delays/pipeline  mask(pipeline){latency=2}
      mask help:
      | An explicitly laid-out delay line to avoid mapping to SRL16s
      | for use in pipelining to help achieve timing closure.
      mask init:
      | pipeline_init(gcb,'latency',latency);
      settings: AttributesFormatString=Latency = %<latency>
      mask Display:
      | port_label('input', 1, 'd');
      | port_label('output', 1, 'q');
      | disp(['Z^-', num2str(latency)]);
  Delay98 : Subsystem  AncestorBlock=casper_library_delays/pipeline  mask(pipeline){latency=2}
      mask help:
      | An explicitly laid-out delay line to avoid mapping to SRL16s
      | for use in pipelining to help achieve timing closure.
      mask init:
      | pipeline_init(gcb,'latency',latency);
      settings: AttributesFormatString=Latency = %<latency>
      mask Display:
      | port_label('input', 1, 'd');
      | port_label('output', 1, 'q');
      | disp(['Z^-', num2str(latency)]);
  Logical{1..4} (4 alike) : xbsIndex_r4/Logical  logical_function=AND  inputs=2  en=off  latency=1  precision=Full  arith_type=Unsigned  n_bits=8  bin_pt=2  align_bp=on  dbl_ovrd=off  block_type=logical
      settings: xl_area=[0, 0, 0, 0, 0, 0, 0]
  Register : xbsIndex_r4/Register  init=0  rst=on  en=on  dbl_ovrd=off  block_type=register
  Slice : xbsIndex_r4/Slice  nbits=16  boolean_output=off  mode=Two Bit Locations  bit1=0  base1=MSB of Input  bit0=xeng_int_bits  base0=LSB of Input  dbl_ovrd=off  block_type=slice
      settings: infoedit="Extracts a given range of bits from each input sample and presents it at the output.  The output type is ordinarily unsigned with binary point at zero, but can be Boolean when the slice is one bit wide.<P><P>Hardware notes: In hardware this block costs nothing."  block_version=10.1.3
  ant_cnt : xbsIndex_r4/Counter  cnt_type=Free Running  cnt_to=1023  operation=Up  start_count=0  cnt_by_val=1  arith_type=Unsigned  n_bits=xeng_int_bits + n_ants_bits  bin_pt=0  load_pin=off  rst=on  en=on  explicit_period=on  period=1  dbl_ovrd=off  use_behavioral_HDL=on  implementation=Fabric  use_rpm=on  block_type=counter
      settings: xl_area=[0, 0, 0, 0, 0, 0, 0]
  sync_ctr1 : xbsIndex_r4/Counter  cnt_type=Free Running  cnt_to=1023  operation=Up  start_count=0  cnt_by_val=1  arith_type=Unsigned  n_bits=32  bin_pt=0  load_pin=off  rst=on  en=on  explicit_period=on  period=1  dbl_ovrd=off  use_behavioral_HDL=on  implementation=Fabric  use_rpm=on  block_type=counter
      settings: xl_area=[0, 0, 0, 0, 0, 0, 0]
  sync_ctr5 : xbsIndex_r4/Counter  cnt_type=Free Running  cnt_to=1023  operation=Up  start_count=0  cnt_by_val=1  arith_type=Unsigned  n_bits=16  bin_pt=0  load_pin=off  rst=on  en=on  explicit_period=on  period=1  dbl_ovrd=off  use_behavioral_HDL=on  implementation=Fabric  use_rpm=on  block_type=counter
      settings: xl_area=[0, 0, 0, 0, 0, 0, 0]
  sync_ctr6 : xbsIndex_r4/Counter  cnt_type=Free Running  cnt_to=1023  operation=Up  start_count=0  cnt_by_val=1  arith_type=Unsigned  n_bits=16  bin_pt=0  load_pin=off  rst=on  en=on  explicit_period=on  period=1  dbl_ovrd=off  use_behavioral_HDL=on  implementation=Fabric  use_rpm=on  block_type=counter
      settings: xl_area=[0, 0, 0, 0, 0, 0, 0]
  sync_ctr8 : xbsIndex_r4/Counter  cnt_type=Free Running  cnt_to=1023  operation=Up  start_count=0  cnt_by_val=1  arith_type=Unsigned  n_bits=32  bin_pt=0  load_pin=off  rst=on  en=on  explicit_period=on  period=1  dbl_ovrd=off  use_behavioral_HDL=on  implementation=Fabric  use_rpm=on  block_type=counter
      settings: xl_area=[0, 0, 0, 0, 0, 0, 0]
  spectr_cnt : Outport
  last_missed_ant : Outport  Port=2
  recv_ctr : Outport  Port=3
  recv_errctr : Outport  Port=4
  timeout_errctr : Outport  Port=5
  pktdisc_errctr : Outport  Port=6
  wires:
  Convert/1 -> last_missed_ant/1
  Delay15/1(q) -> Convert/1
  Delay11/1(q) -> spectr_cnt/1
  Delay10/1(q) -> recv_ctr/1
  [reord_recverr1] -> Delay9/1(d)
  [reord_valid1] -> Delay3/1(d)
  [reord_sync1] -> Delay2/1(d)
  [cnt_rst] -> Delay1/1(d)
  [reord_recverr1] -> Delay7/1(d)
  Delay7/1(q) -> Logical2/2
  Logical2/1 -> sync_ctr1/2
  Delay6/1(q) -> pktdisc_errctr/1
  Delay5/1(q) -> timeout_errctr/1
  Delay4/1(q) -> recv_errctr/1
  sync_ctr1/1 -> Delay4/1(d)
  sync_ctr5/1 -> Delay6/1(d)
  sync_ctr6/1 -> Delay5/1(d)
  [reord_recv1] -> Delay13/1(d)
  Delay14/1(q) -> Logical4/1
  [reord_valid1] -> Delay14/1(d)
  [cnt_rst] -> Delay12/1(d)
  Delay13/1(q) -> Logical4/2
  Delay12/1(q) -> sync_ctr8/1
  Logical4/1 -> sync_ctr8/2
  sync_ctr8/1 -> Delay10/1(d)
  [reord_pktdisc1] -> Delay8/1(d)
  Delay8/1(q) -> Logical1/2
  Logical1/1 -> sync_ctr5/2
  Delay98/1(q) -> Logical3/1, Logical1/1, Logical2/1
  [reord_valid1] -> Delay98/1(d)
  [cnt_rst] -> Delay96/1(d)
  Delay97/1(q) -> Logical3/2
  Delay96/1(q) -> sync_ctr6/1, sync_ctr5/1, sync_ctr1/1
  Logical3/1 -> sync_ctr6/2
  [reord_timeouterr1] -> Delay97/1(d)
  Delay9/1(q) -> Register/3
  Slice/1 -> Register/1
  ant_cnt/1 -> Slice/1
  Register/1 -> Delay15/1(d)
  Counter1/1 -> Delay11/1(d)
  Delay2/1(q) -> ant_cnt/1, Counter1/2
  Delay3/1(q) -> ant_cnt/2
  Delay1/1(q) -> Register/2, Counter1/1
